simulink model "lab3test"  (R2025a)
settings: Solver=VariableStepAuto  StartTime=0.0  StopTime=10.0  RelTol=1e-3
settings Model: Creator=isaki  LastModifiedBy=isaki

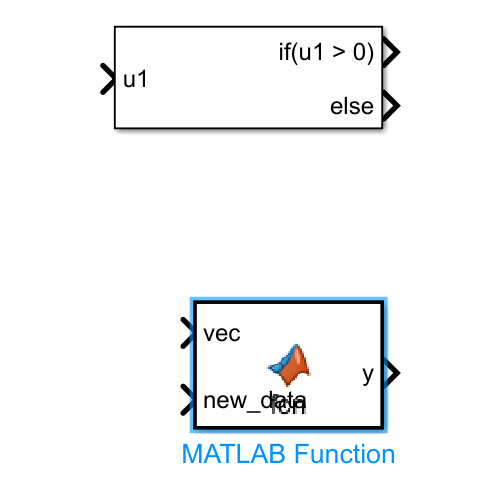
[thumbnail: Simulink's stored preview of the top-level diagram]
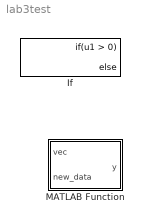
== system lab3test ==
  If : If
  MATLAB Function : MATLAB Function  TreatAsAtomicUnit=on

== matlab function lab3test/MATLAB Function ==
  data: vec input; y output; new_data input
function y = fcn(vec, new_data)
    % Declare a persistent variable to hold the last valid value
    persistent last_val;
    
    % Initialize the persistent variable if empty
    if isempty(last_val)
        last_val = 0; 
    end
    
    % Update value if input is not zero
    if new_data ~= 0
        last_val = vec;
    end
    
    % Output the current valid or retained last value
y = last_val;
